simulink model "SimplePropellerModel"  (R2026b)
settings: Solver=VariableStepAuto  StopTime=10
undefined symbols (not defined in the file or in its folder): Epsilon, magnitude
settings Model: Creator=esmithzb  LastModifiedBy=Ninad
settings DebuggingCC: MergeDetectMultiDrivingBlocksExec=none  UnderspecifiedInitializationDetection=Classic
settings ModelReferenceCC: PropagateSignalLabelsOutOfModel=off
settings RTWCC: GPUComputeCapability=5.0

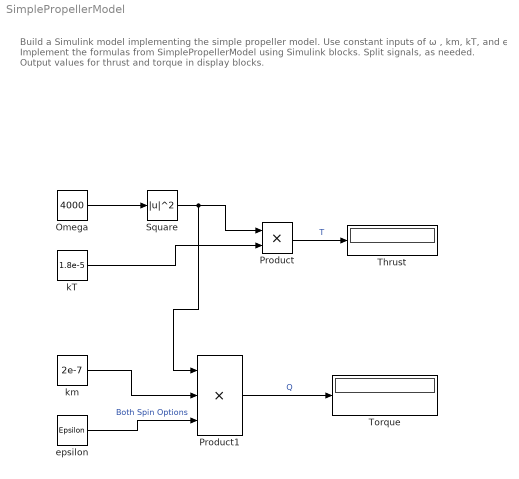
== system SimplePropellerModel ==
  note: Build a Simulink model implementing the simple propeller model.
      | Use constant inputs of ω , km, kT, and ϵ
      | Implement the formulas from SimplePropellerModel using Simulink blocks. Split signals, as needed.
      | Output values for thrust and torque in display blocks.
  Omega : Constant  Value=4000
  Product : Product
  Product1 : Product  Inputs=3
  Square : Math  Operator=magnitude^2  OutputSignalType=real
  Thrust : Display
  Torque : Display
  epsilon : Constant  Value=Epsilon
  kT : Constant  Value=1.8e-5
  km : Constant  Value=2e-7
  wires:
  Omega/1 -> Square/1
  Square/1 -> Product1/1, Product/1
  kT/1 -> Product/2
  Product/1 -> Thrust/1  "T"
  km/1 -> Product1/2
  epsilon/1 -> Product1/3  "Both Spin Options"
  Product1/1 -> Torque/1  "Q"
